simulink model "rolling_contact_test"  (R2026b)
settings: Solver=VariableStepAuto  StopTime=5
undefined symbols (not defined in the file): f_rr, k_contact, k_gx, k_gy, k_x, m_body, m_wheel, miu_p, miu_s, mu_slide, mu_stick, omega_rr_eps, r_wheel, sgn, v_c_max, v_gx_max, v_gy_max, vLimit, X, Y, Z
libraries: nesl_utility x19, sm_lib x18, simulink x7, simulink_extras x1
settings Model: Creator=h4nty  LastModifiedBy=h4nty
settings RTWCC: GPUComputeCapability=5.0
settings SimscapeCC: SimscapeUseEnergyAccounting=off

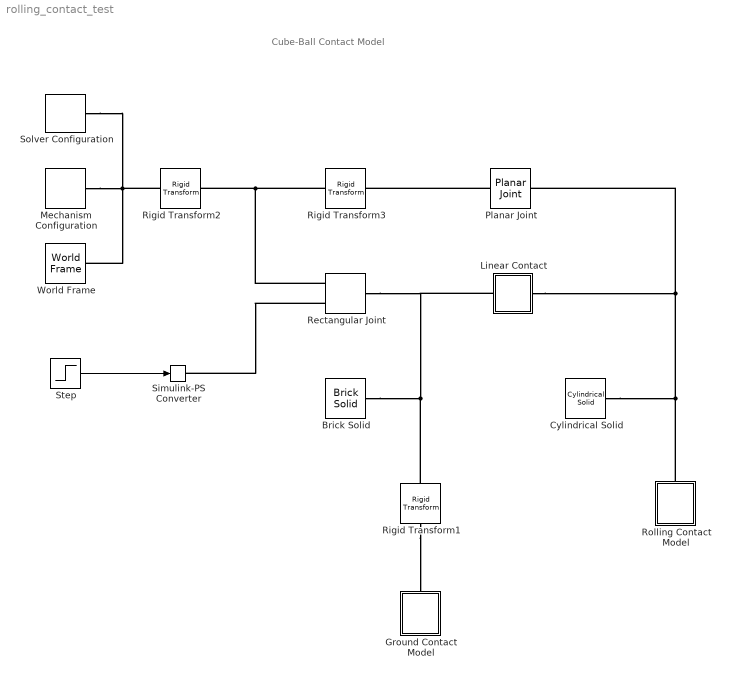
== system rolling_contact_test ==
  note: Cube-Ball Contact Model
  Brick Solid : sm_lib/Body Elements/Brick Solid  BrickDimensions=[1 1 1 ]  BrickDimensionsUnits=m  ExportEntireGeometry=off  InertiaType=CalculateFromGeometry  BasedOnType=Mass  Density=1000  DensityUnits=kg/m^3  Mass=m_body  MassUnits=kg  CenterOfMass=[0 0 0]  CenterOfMassUnits=m  MomentsOfInertia=[1 1 1]  MomentsOfInertiaUnits=kg*m^2  ProductsOfInertia=[0 0 0]  ProductsOfInertiaUnits=kg*m^2  GraphicType=FromGeometry  MarkerShape=Sphere  MarkerSize=10  GraphicVisPropType=SimpleVisualProperties  GraphicDiffuseColor=[0.5 0.5 0.5]  GraphicOpacity=1  GraphicSpecularColor=[0.5 0.5 0.5 1.0]  GraphicAmbientColor=[0.15 0.15 0.15 1.0]  GraphicEmissiveColor=[0.0 0.0 0.0 1.0]  GraphicShininess=75  DoExposeReferenceFrame=on  SerializedFrames=<Frames/>
  Cylindrical Solid : sm_lib/Body Elements/Cylindrical Solid  CylinderRadius=0.5  CylinderRadiusUnits=m  CylinderLength=1  CylinderLengthUnits=m  ExportEntireGeometry=off  InertiaType=CalculateFromGeometry  BasedOnType=Mass  Density=1000  DensityUnits=kg/m^3  Mass=m_wheel  MassUnits=kg  CenterOfMass=[0 0 0]  CenterOfMassUnits=m  MomentsOfInertia=[1 1 1]  MomentsOfInertiaUnits=kg*m^2  ProductsOfInertia=[0 0 0]  ProductsOfInertiaUnits=kg*m^2  GraphicType=FromGeometry  MarkerShape=Sphere  MarkerSize=10  GraphicVisPropType=SimpleVisualProperties  GraphicDiffuseColor=[0.5 0.5 0.5]  GraphicOpacity=1  GraphicSpecularColor=[0.5 0.5 0.5 1.0]  GraphicAmbientColor=[0.15 0.15 0.15 1.0]  GraphicEmissiveColor=[0.0 0.0 0.0 1.0]  GraphicShininess=75  DoExposeReferenceFrame=on  SerializedFrames=<Frames/>
  Ground Contact Model : Subsystem
  Linear Contact : Subsystem
  Mechanism Configuration : sm_lib/Utilities/Mechanism Configuration  UniformGravity=Constant  GravityVector=[0 -9.80665 0]  GravityVectorUnits=m/s^2  LinearizationDelta=0.001  JointModeTransitionNonlinearIterations=2
  Planar Joint : sm_lib/Joints/Planar Joint  JointMode=Normal  CompositeWrenchDir=FollowerOnBase  CompositeWrenchFrame=BaseFrame  SenseConstraintForce=off  SenseConstraintTorque=off  SenseTotalForce=off  SenseTotalTorque=off  PxPositionTargetSpecify=off  PxPositionTargetPriority=High  PxPositionTargetValue=0  PxPositionTargetValueUnits=m  PxVelocityTargetSpecify=off  PxVelocityTargetPriority=High  PxVelocityTargetValue=0  PxVelocityTargetValueUnits=m/s  PxEquilibriumPosition=0  PxEquilibriumPositionUnits=m  PxSpringStiffness=0  PxSpringStiffnessUnits=N/m  PxDampingCoefficient=0  PxDampingCoefficientUnits=N/(m/s)  PxLowerLimitSpecify=off  PxLowerLimitBound=-1  PxLowerLimitBoundUnits=m  PxLowerLimitStiffness=1e6  PxLowerLimitStiffnessUnits=N/m  PxLowerLimitDamping=1e3  PxLowerLimitDampingUnits=N/(m/s)  PxLowerLimitTransitionRegionWidth=1e-4  PxLowerLimitTransitionRegionWidthUnits=m  PxUpperLimitSpecify=off  PxUpperLimitBound=1  PxUpperLimitBoundUnits=m  PxUpperLimitStiffness=1e6  PxUpperLimitStiffnessUnits=N/m  PxUpperLimitDamping=1e3  PxUpperLimitDampingUnits=N/(m/s)  PxUpperLimitTransitionRegionWidth=1e-4  PxUpperLimitTransitionRegionWidthUnits=m  PxTorqueActuationMode=NoTorque  PxMotionActuationMode=ComputedMotion  PxSensePosition=off  PxSenseVelocity=off  PxSenseAcceleration=off  PxSenseTorqueForce=off  PxSenseLowerLimitTorqueForce=off  PxSenseUpperLimitTorqueForce=off  PyPositionTargetSpecify=off  PyPositionTargetPriority=High  PyPositionTargetValue=0  PyPositionTargetValueUnits=m  PyVelocityTargetSpecify=off  PyVelocityTargetPriority=High  PyVelocityTargetValue=0  PyVelocityTargetValueUnits=m/s  PyEquilibriumPosition=0  PyEquilibriumPositionUnits=m  PySpringStiffness=0  PySpringStiffnessUnits=N/m  PyDampingCoefficient=0  PyDampingCoefficientUnits=N/(m/s)  PyLowerLimitSpecify=off  PyLowerLimitBound=-1  PyLowerLimitBoundUnits=m  PyLowerLimitStiffness=1e6  PyLowerLimitStiffnessUnits=N/m  PyLowerLimitDamping=1e3  PyLowerLimitDampingUnits=N/(m/s)  PyLowerLimitTransitionRegionWidth=1e-4  PyLowerLimitTransitionRegionWidthUnits=m  PyUpperLimitSpecify=off  PyUpperLimitBound=1  PyUpperLimitBoundUnits=m  PyUpperLimitStiffness=1e6  PyUpperLimitStiffnessUnits=N/m  PyUpperLimitDamping=1e3  PyUpperLimitDampingUnits=N/(m/s)  PyUpperLimitTransitionRegionWidth=1e-4  PyUpperLimitTransitionRegionWidthUnits=m  PyTorqueActuationMode=NoTorque  PyMotionActuationMode=ComputedMotion  PySensePosition=off  PySenseVelocity=off  PySenseAcceleration=off  PySenseTorqueForce=off  PySenseLowerLimitTorqueForce=off  PySenseUpperLimitTorqueForce=off  RzPositionTargetSpecify=off  RzPositionTargetPriority=High  RzPositionTargetValue=0  RzPositionTargetValueUnits=deg  RzVelocityTargetSpecify=off  RzVelocityTargetPriority=High  RzVelocityTargetValue=0  RzVelocityTargetValueUnits=deg/s  RzEquilibriumPosition=0  RzEquilibriumPositionUnits=deg  RzSpringStiffness=0  RzSpringStiffnessUnits=N*m/deg  RzDampingCoefficient=0  RzDampingCoefficientUnits=N*m/(deg/s)  RzLowerLimitSpecify=off  RzLowerLimitBound=-90  RzLowerLimitBoundUnits=deg  RzLowerLimitStiffness=1e4  RzLowerLimitStiffnessUnits=N*m/deg  RzLowerLimitDamping=10  RzLowerLimitDampingUnits=N*m/(deg/s)  RzLowerLimitTransitionRegionWidth=0.1  RzLowerLimitTransitionRegionWidthUnits=deg  RzUpperLimitSpecify=off  RzUpperLimitBound=90  RzUpperLimitBoundUnits=deg  RzUpperLimitStiffness=1e4  RzUpperLimitStiffnessUnits=N*m/deg  RzUpperLimitDamping=10  RzUpperLimitDampingUnits=N*m/(deg/s)  RzUpperLimitTransitionRegionWidth=0.1  RzUpperLimitTransitionRegionWidthUnits=deg  RzTorqueActuationMode=NoTorque  RzMotionActuationMode=ComputedMotion  RzSensePosition=off  RzSenseVelocity=off  RzSenseAcceleration=off  RzSenseTorqueForce=off  RzSenseLowerLimitTorqueForce=off  RzSenseUpperLimitTorqueForce=off
  Rectangular Joint : sm_lib/Joints/Rectangular Joint  JointMode=Normal  CompositeWrenchDir=FollowerOnBase  CompositeWrenchFrame=BaseFrame  SenseConstraintForce=off  SenseConstraintTorque=off  SenseTotalForce=off  SenseTotalTorque=off  PxPositionTargetSpecify=off  PxPositionTargetPriority=High  PxPositionTargetValue=0  PxPositionTargetValueUnits=m  PxVelocityTargetSpecify=off  PxVelocityTargetPriority=High  PxVelocityTargetValue=0  PxVelocityTargetValueUnits=m/s  PxEquilibriumPosition=0  PxEquilibriumPositionUnits=m  PxSpringStiffness=0  PxSpringStiffnessUnits=N/m  PxDampingCoefficient=0  PxDampingCoefficientUnits=N/(m/s)  PxLowerLimitSpecify=off  PxLowerLimitBound=-1  PxLowerLimitBoundUnits=m  PxLowerLimitStiffness=1e6  PxLowerLimitStiffnessUnits=N/m  PxLowerLimitDamping=1e3  PxLowerLimitDampingUnits=N/(m/s)  PxLowerLimitTransitionRegionWidth=1e-4  PxLowerLimitTransitionRegionWidthUnits=m  PxUpperLimitSpecify=off  PxUpperLimitBound=1  PxUpperLimitBoundUnits=m  PxUpperLimitStiffness=1e6  PxUpperLimitStiffnessUnits=N/m  PxUpperLimitDamping=1e3  PxUpperLimitDampingUnits=N/(m/s)  PxUpperLimitTransitionRegionWidth=1e-4  PxUpperLimitTransitionRegionWidthUnits=m  PxTorqueActuationMode=InputTorque  PxMotionActuationMode=ComputedMotion  PxSensePosition=off  PxSenseVelocity=off  PxSenseAcceleration=off  PxSenseTorqueForce=off  PxSenseLowerLimitTorqueForce=off  PxSenseUpperLimitTorqueForce=off  PyPositionTargetSpecify=off  PyPositionTargetPriority=High  PyPositionTargetValue=0  PyPositionTargetValueUnits=m  PyVelocityTargetSpecify=off  PyVelocityTargetPriority=High  PyVelocityTargetValue=0  PyVelocityTargetValueUnits=m/s  PyEquilibriumPosition=0  PyEquilibriumPositionUnits=m  PySpringStiffness=0  PySpringStiffnessUnits=N/m  PyDampingCoefficient=0  PyDampingCoefficientUnits=N/(m/s)  PyLowerLimitSpecify=off  PyLowerLimitBound=-1  PyLowerLimitBoundUnits=m  PyLowerLimitStiffness=1e6  PyLowerLimitStiffnessUnits=N/m  PyLowerLimitDamping=1e3  PyLowerLimitDampingUnits=N/(m/s)  PyLowerLimitTransitionRegionWidth=1e-4  PyLowerLimitTransitionRegionWidthUnits=m  PyUpperLimitSpecify=off  PyUpperLimitBound=1  PyUpperLimitBoundUnits=m  PyUpperLimitStiffness=1e6  PyUpperLimitStiffnessUnits=N/m  PyUpperLimitDamping=1e3  PyUpperLimitDampingUnits=N/(m/s)  PyUpperLimitTransitionRegionWidth=1e-4  PyUpperLimitTransitionRegionWidthUnits=m  PyTorqueActuationMode=NoTorque  PyMotionActuationMode=ComputedMotion  PySensePosition=off  PySenseVelocity=off  PySenseAcceleration=off  PySenseTorqueForce=off  PySenseLowerLimitTorqueForce=off  PySenseUpperLimitTorqueForce=off
  Rigid Transform1 : sm_lib/Frames and Transforms/Rigid Transform  RotationMethod=None  FollAlignAxisA=+X  BaseAlignAxisA=+Y  FollAlignAxisB=+Y  BaseAlignAxisB=+Z  RotationStandardAxis=+Y  RotationAngle=-90  RotationAngleUnits=deg  RotationArbitraryAxis=[0 0 1]  RotationSequenceAxes=FollowerAxes  RotationSequence=XYX  RotationSequenceAngles=[0 0 0]  RotationSequenceAnglesUnits=deg  RotationMatrix=[1 0 0; 0 1 0; 0 0 1]  Quaternion=[1 0 0 0]  TranslationMethod=Cartesian  TranslationCartesianOffset=[0 -0.5 0]  TranslationCartesianOffsetUnits=m  TranslationStandardAxis=+X  TranslationStandardOffset=+0.5  TranslationStandardOffsetUnits=m  TranslationROffset=r_ball  TranslationROffsetUnits=m  TranslationThetaOffset=0  TranslationThetaOffsetUnits=deg  TranslationZOffset=0  TranslationZOffsetUnits=m
  Rigid Transform2 : sm_lib/Frames and Transforms/Rigid Transform  RotationMethod=None  FollAlignAxisA=+X  BaseAlignAxisA=+Y  FollAlignAxisB=+Y  BaseAlignAxisB=+Z  RotationStandardAxis=+Y  RotationAngle=90  RotationAngleUnits=deg  RotationArbitraryAxis=[0 0 1]  RotationSequenceAxes=FollowerAxes  RotationSequence=XYX  RotationSequenceAngles=[0 0 0]  RotationSequenceAnglesUnits=deg  RotationMatrix=[1 0 0; 0 1 0; 0 0 1]  Quaternion=[1 0 0 0]  TranslationMethod=Cartesian  TranslationCartesianOffset=[0 +0.5 0]  TranslationCartesianOffsetUnits=m  TranslationStandardAxis=+X  TranslationStandardOffset=+0.5  TranslationStandardOffsetUnits=m  TranslationROffset=r_ball  TranslationROffsetUnits=m  TranslationThetaOffset=0  TranslationThetaOffsetUnits=deg  TranslationZOffset=0  TranslationZOffsetUnits=m
  Rigid Transform3 : sm_lib/Frames and Transforms/Rigid Transform  RotationMethod=None  FollAlignAxisA=+X  BaseAlignAxisA=+Y  FollAlignAxisB=+Y  BaseAlignAxisB=+Z  RotationStandardAxis=+Y  RotationAngle=90  RotationAngleUnits=deg  RotationArbitraryAxis=[0 0 1]  RotationSequenceAxes=FollowerAxes  RotationSequence=XYX  RotationSequenceAngles=[0 0 0]  RotationSequenceAnglesUnits=deg  RotationMatrix=[1 0 0; 0 1 0; 0 0 1]  Quaternion=[1 0 0 0]  TranslationMethod=Cartesian  TranslationCartesianOffset=[2 0 0]  TranslationCartesianOffsetUnits=m  TranslationStandardAxis=+X  TranslationStandardOffset=+0.5  TranslationStandardOffsetUnits=m  TranslationROffset=r_ball  TranslationROffsetUnits=m  TranslationThetaOffset=0  TranslationThetaOffsetUnits=deg  TranslationZOffset=0  TranslationZOffsetUnits=m
  Rolling Contact Model : Subsystem
  Simulink-PS Converter : nesl_utility/Simulink-PS Converter  PhysicalDomain=network_engine_domain  SubClassName=ps_input  LeftPortType=input  RightPortType=output  PseudoPeriodic=off  Frequencies=[]  NoiseDistribution=none  NoiseParameters=[]  Unit=N  AffineConversion=off  FilteringAndDerivatives=provide  SimscapeFilterOrder=1  InputFilterTimeConstant=0.001  UdotUserProvided=0
  Solver Configuration : nesl_utility/Solver Configuration  PhysicalDomain=network_engine_domain  SubClassName=solver  LeftPortType=input  RightPortType=generic  Tones=[]  Harmonics=[]  SimulateNoise=off  Profile=off  UseLocalSampling=off  EnableSwitchedLinearOptims=on  FrequencyDomain=off  UseCCode=off  RelTol=0.001  AbsTol=0.001  MinStep=1e-09  ToWorkspace=off  RevertToSquareIcSolve=off  NumHomotopyIterations=100  PhasorMode=off  PhasorModeNumHarmonics=1  ConsistencySolver=NEWTON_FTOL  CanonicalOrdering=UNORDERED  OptimizeIntermediates=UNOPTIMIZED  MulticoreSolverChoice=BACKWARD_EULER  IndexReductionMethod=DerivativeReplacement  DoDC=off  ResidualTolerance=1e-09  ConsistencyTolSource=GLOBAL  ConsistencyAbsTol=0.001  ConsistencyRelTol=0.001  ConsistencyTolFactor=0.001  UseLocalSolver=off  LocalSolverChoice=NE_BACKWARD_EULER_ADVANCER  ResolveIndetEquations=on  FunctionEvalNumThread=1  LocalSolverSampleTime=0.001  DoFixedCost=off  MaxNonlinIter=3  MaxModeIter=2  ComputeImpulses=off  ImpulseIterations=2  LinearAlgebra=auto  LinearAlgebraNumThread=0  EquationFormulation=NE_TIME_EF  DelaysMemoryBudget=1024  AutomaticFiltering=on  FilteringTimeConstant=0.001  PartitionStorageMethod=AS_NEEDED  PartitionMemoryBudget=1024  PartitionMethod=BALANCED  MultibodyUseLocalSolver=off  MultibodyLocalSolverChoice=ODE1  MultibodyLocalSolverSampleTime=0.001
  Step : Step  InitialValue=100  FinalValue=0  SampleTime=0
  "World Frame " : sm_lib/Frames and Transforms/World Frame
  wires:
  Step/1 -> Simulink-PS Converter/1
  connections:
  Rigid Transform1/RConn1 -- Ground Contact Model/LConn1
  Solver Configuration/RConn1 -- "World Frame "/RConn1 -- Rigid Transform2/LConn1 -- Mechanism Configuration/RConn1
  Rectangular Joint/LConn1 -- Rigid Transform3/LConn1 -- Rigid Transform2/RConn1
  Rigid Transform1/LConn1 -- Linear Contact/LConn1 -- Rectangular Joint/RConn1 -- Brick Solid/RConn1
  Rectangular Joint/LConn2 -- Simulink-PS Converter/RConn1
  Planar Joint/LConn1 -- Rigid Transform3/RConn1
  Rolling Contact Model/LConn1 -- Cylindrical Solid/RConn1 -- Linear Contact/RConn1 -- Planar Joint/RConn1

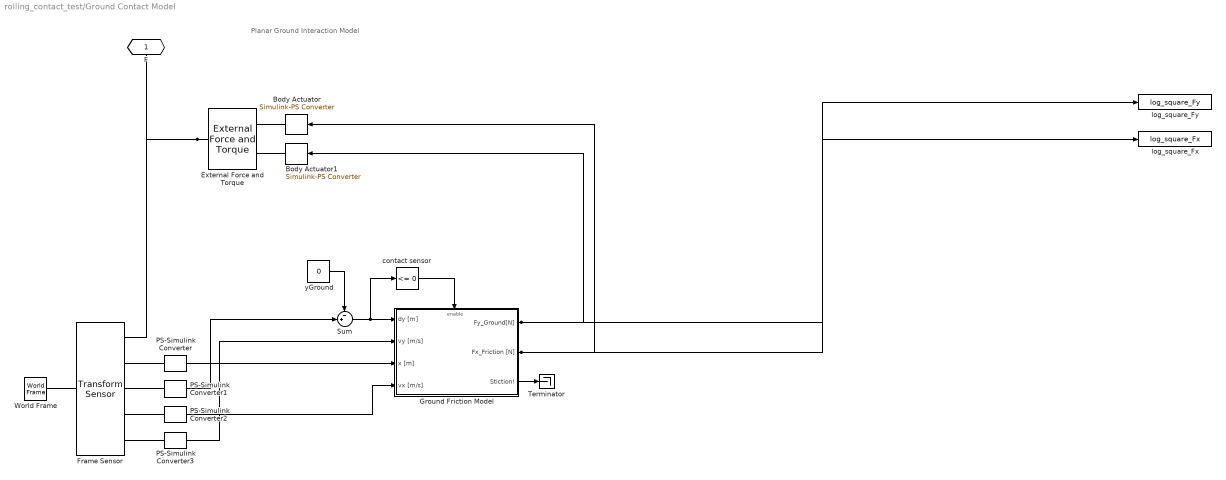
== system rolling_contact_test/Ground Contact Model ==
  note: Planar Ground Interaction Model
  " Body Actuator" : nesl_utility/Simulink-PS Converter  PhysicalDomain=network_engine_domain  SubClassName=ps_input  LeftPortType=input  RightPortType=output  PseudoPeriodic=off  Frequencies=[]  NoiseDistribution=none  NoiseParameters=[]  Unit=N  AffineConversion=off  FilteringAndDerivatives=zero  SimscapeFilterOrder=1  InputFilterTimeConstant=.001  UdotUserProvided=0
  " Body Actuator1" : nesl_utility/Simulink-PS Converter  PhysicalDomain=network_engine_domain  SubClassName=ps_input  LeftPortType=input  RightPortType=output  PseudoPeriodic=off  Frequencies=[]  NoiseDistribution=none  NoiseParameters=[]  Unit=N  AffineConversion=off  FilteringAndDerivatives=zero  SimscapeFilterOrder=1  InputFilterTimeConstant=.001  UdotUserProvided=0
  External Force and Torque : sm_lib/Forces and Torques/External Force and Torque  EnableForceX=on  EnableForceY=on  EnableForceZ=off  EnableForce=off  ForceResolutionFrame=World  EnableTorqueX=off  EnableTorqueY=off  EnableTorqueZ=off  EnableTorque=off  TorqueResolutionFrame=AttachedFrame
  Frame Sensor : sm_lib/Frames and Transforms/Transform Sensor  ObservationFrame=World  ExpressedInFrame=World  RotationSequence=XYX  SenseAngle=off  SenseAxis=off  SenseQ=off  SenseR=off  SenseRotationSequence=off  SenseOmegaX=off  SenseOmegaY=off  SenseOmegaZ=off  SenseOmega=off  SenseQDot=off  SenseRDot=off  SenseRotationSequenceDot=off  SenseAlphaX=off  SenseAlphaY=off  SenseAlphaZ=off  SenseAlpha=off  SenseQDDot=off  SenseRDDot=off  SenseX=on  SenseY=on  SenseZ=off  SenseXYZ=off  SenseRad=off  SenseAzim=off  SenseDist=off  SenseInc=off  SenseXDot=on  SenseYDot=on  SenseZDot=off  SenseXYZDot=off  SenseRadDot=off  SenseAzimDot=off  SenseDistDot=off  SenseIncDot=off  SenseXDDot=off  SenseYDDot=off  SenseZDDot=off  SenseXYZDDot=off  SenseRadDDot=off  SenseAzimDDot=off  SenseDistDDot=off  SenseIncDDot=off
  Ground Friction Model : Subsystem
  PS-Simulink Converter : nesl_utility/PS-Simulink Converter  PhysicalDomain=network_engine_domain  SubClassName=ps_output  LeftPortType=input  RightPortType=output  PseudoPeriodic=off  Frequencies=[]  VectorFormat=1-D array  Unit=m  AffineConversion=off
  PS-Simulink Converter1 : nesl_utility/PS-Simulink Converter  PhysicalDomain=network_engine_domain  SubClassName=ps_output  LeftPortType=input  RightPortType=output  PseudoPeriodic=off  Frequencies=[]  VectorFormat=1-D array  Unit=m  AffineConversion=off
  PS-Simulink Converter2 : nesl_utility/PS-Simulink Converter  PhysicalDomain=network_engine_domain  SubClassName=ps_output  LeftPortType=input  RightPortType=output  PseudoPeriodic=off  Frequencies=[]  VectorFormat=1-D array  Unit=m/s  AffineConversion=off
  PS-Simulink Converter3 : nesl_utility/PS-Simulink Converter  PhysicalDomain=network_engine_domain  SubClassName=ps_output  LeftPortType=input  RightPortType=output  PseudoPeriodic=off  Frequencies=[]  VectorFormat=1-D array  Unit=m/s  AffineConversion=off
  Sum : Sum  Inputs=-+|
  Terminator : Terminator
  World Frame : sm_lib/Frames and Transforms/World Frame
  contact sensor : simulink/Logic and Bit Operations/Compare To Zero  relop=<=  OutDataTypeStr=boolean
  log_square_Fx : ToWorkspace  VariableName=log_square_Fx  SaveFormat=Timeseries  SampleTime=-1
  log_square_Fy : ToWorkspace  VariableName=log_square_Fy  SaveFormat=Timeseries  SampleTime=-1
  yGround : Constant  Value=0
  F : PMIOPort  Side=Left
  wires:
  PS-Simulink Converter2/1 -> Ground Friction Model/4(vx [m/s])
  PS-Simulink Converter/1 -> Ground Friction Model/3(x [m])
  PS-Simulink Converter3/1 -> Ground Friction Model/2(vy [m/s])
  PS-Simulink Converter1/1 -> Sum/2
  Sum/1 -> contact sensor/1, Ground Friction Model/1(dy [m])
  yGround/1 -> Sum/1
  contact sensor/1 -> Ground Friction Model/Enable
  Ground Friction Model/1(Fy_Ground[N]) -> " Body Actuator1"/1, log_square_Fy/1
  Ground Friction Model/2(Fx_Friction [N]) -> " Body Actuator"/1, log_square_Fx/1
  Ground Friction Model/3(Stiction!) -> Terminator/1
  connections:
  World Frame/RConn1 -- Frame Sensor/LConn1
  PS-Simulink Converter2/LConn1 -- Frame Sensor/RConn4
  PS-Simulink Converter1/LConn1 -- Frame Sensor/RConn3
  Frame Sensor/RConn2 -- PS-Simulink Converter/LConn1
  PS-Simulink Converter3/LConn1 -- Frame Sensor/RConn5
  External Force and Torque/RConn1 -- Frame Sensor/RConn1 -- F/RConn1
  External Force and Torque/LConn2 -- " Body Actuator1"/RConn1
  External Force and Torque/LConn1 -- " Body Actuator"/RConn1

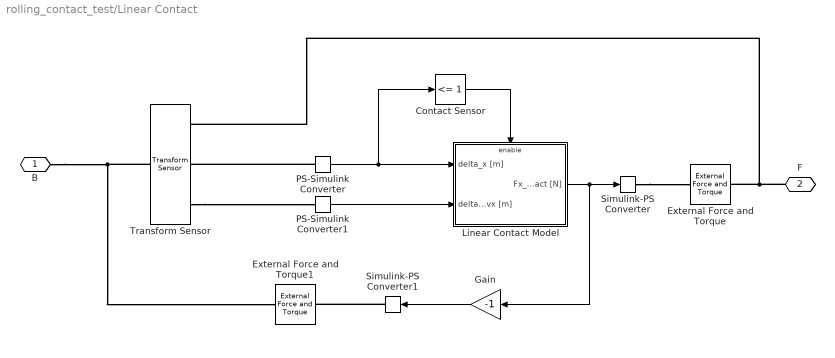
== system rolling_contact_test/Linear Contact ==
  Contact Sensor : simulink/Logic and Bit Operations/Compare To Constant  relop=<=  const=1  OutDataTypeStr=boolean  ZeroCross=off
  External Force and Torque : sm_lib/Forces and Torques/External Force and Torque  EnableForceX=on  EnableForceY=off  EnableForceZ=off  EnableForce=off  ForceResolutionFrame=AttachedFrame  EnableTorqueX=off  EnableTorqueY=off  EnableTorqueZ=off  EnableTorque=off  TorqueResolutionFrame=AttachedFrame
  External Force and Torque1 : sm_lib/Forces and Torques/External Force and Torque  EnableForceX=on  EnableForceY=off  EnableForceZ=off  EnableForce=off  ForceResolutionFrame=AttachedFrame  EnableTorqueX=off  EnableTorqueY=off  EnableTorqueZ=off  EnableTorque=off  TorqueResolutionFrame=AttachedFrame
  Gain : Gain  Gain=-1
  Linear Contact Model : Subsystem
  PS-Simulink Converter : nesl_utility/PS-Simulink Converter  PhysicalDomain=network_engine_domain  SubClassName=ps_output  LeftPortType=input  RightPortType=output  PseudoPeriodic=off  Frequencies=[]  VectorFormat=inherit  Unit=inherit  AffineConversion=off
  PS-Simulink Converter1 : nesl_utility/PS-Simulink Converter  PhysicalDomain=network_engine_domain  SubClassName=ps_output  LeftPortType=input  RightPortType=output  PseudoPeriodic=off  Frequencies=[]  VectorFormat=inherit  Unit=inherit  AffineConversion=off
  Simulink-PS Converter : nesl_utility/Simulink-PS Converter  PhysicalDomain=network_engine_domain  SubClassName=ps_input  LeftPortType=input  RightPortType=output  PseudoPeriodic=off  Frequencies=[]  NoiseDistribution=none  NoiseParameters=[]  Unit=1  AffineConversion=off  FilteringAndDerivatives=provide  SimscapeFilterOrder=1  InputFilterTimeConstant=0.001  UdotUserProvided=0
  Simulink-PS Converter1 : nesl_utility/Simulink-PS Converter  PhysicalDomain=network_engine_domain  SubClassName=ps_input  LeftPortType=input  RightPortType=output  PseudoPeriodic=off  Frequencies=[]  NoiseDistribution=none  NoiseParameters=[]  Unit=1  AffineConversion=off  FilteringAndDerivatives=provide  SimscapeFilterOrder=1  InputFilterTimeConstant=0.001  UdotUserProvided=0
  Transform Sensor : sm_lib/Frames and Transforms/Transform Sensor  ObservationFrame=World  ExpressedInFrame=World  RotationSequence=XYX  SenseAngle=off  SenseAxis=off  SenseQ=off  SenseR=off  SenseRotationSequence=off  SenseOmegaX=off  SenseOmegaY=off  SenseOmegaZ=off  SenseOmega=off  SenseQDot=off  SenseRDot=off  SenseRotationSequenceDot=off  SenseAlphaX=off  SenseAlphaY=off  SenseAlphaZ=off  SenseAlpha=off  SenseQDDot=off  SenseRDDot=off  SenseX=on  SenseY=off  SenseZ=off  SenseXYZ=off  SenseRad=off  SenseAzim=off  SenseDist=off  SenseInc=off  SenseXDot=on  SenseYDot=off  SenseZDot=off  SenseXYZDot=off  SenseRadDot=off  SenseAzimDot=off  SenseDistDot=off  SenseIncDot=off  SenseXDDot=off  SenseYDDot=off  SenseZDDot=off  SenseXYZDDot=off  SenseRadDDot=off  SenseAzimDDot=off  SenseDistDDot=off  SenseIncDDot=off
  B : PMIOPort  Side=Left
  F : PMIOPort  Port=2  Side=Right
  wires:
  PS-Simulink Converter/1 -> Linear Contact Model/1(delta_x [m]), Contact Sensor/1
  Contact Sensor/1 -> Linear Contact Model/Enable
  PS-Simulink Converter1/1 -> Linear Contact Model/2(delta_vx [m])
  Linear Contact Model/1(Fx_contact [N]) -> Gain/1, Simulink-PS Converter/1
  Gain/1 -> Simulink-PS Converter1/1
  connections:
  PS-Simulink Converter/LConn1 -- Transform Sensor/RConn2
  F/RConn1 -- Transform Sensor/RConn1 -- External Force and Torque/RConn1
  Transform Sensor/LConn1 -- B/RConn1 -- External Force and Torque1/RConn1
  Simulink-PS Converter/RConn1 -- External Force and Torque/LConn1
  Transform Sensor/RConn3 -- PS-Simulink Converter1/LConn1
  Simulink-PS Converter1/RConn1 -- External Force and Torque1/LConn1

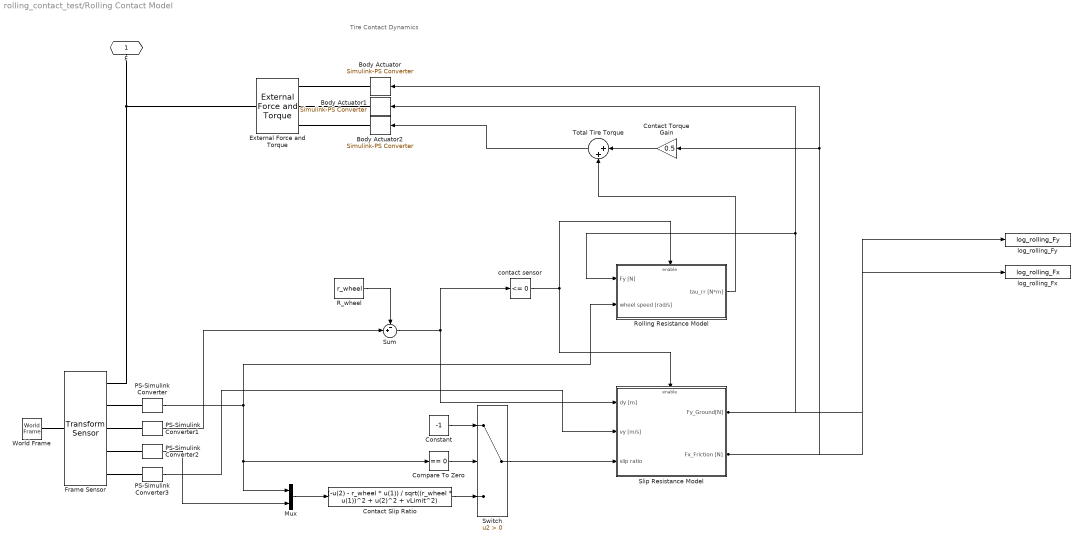
== system rolling_contact_test/Rolling Contact Model ==
  note: Tire Contact Dynamics
  " Body Actuator" : nesl_utility/Simulink-PS Converter  PhysicalDomain=network_engine_domain  SubClassName=ps_input  LeftPortType=input  RightPortType=output  PseudoPeriodic=off  Frequencies=[]  NoiseDistribution=none  NoiseParameters=[]  Unit=N  AffineConversion=off  FilteringAndDerivatives=zero  SimscapeFilterOrder=1  InputFilterTimeConstant=.001  UdotUserProvided=0
  " Body Actuator1" : nesl_utility/Simulink-PS Converter  PhysicalDomain=network_engine_domain  SubClassName=ps_input  LeftPortType=input  RightPortType=output  PseudoPeriodic=off  Frequencies=[]  NoiseDistribution=none  NoiseParameters=[]  Unit=N  AffineConversion=off  FilteringAndDerivatives=zero  SimscapeFilterOrder=1  InputFilterTimeConstant=.001  UdotUserProvided=0
  " Body Actuator2" : nesl_utility/Simulink-PS Converter  PhysicalDomain=network_engine_domain  SubClassName=ps_input  LeftPortType=input  RightPortType=output  PseudoPeriodic=off  Frequencies=[]  NoiseDistribution=none  NoiseParameters=[]  Unit=N*m  AffineConversion=off  FilteringAndDerivatives=zero  SimscapeFilterOrder=1  InputFilterTimeConstant=.001  UdotUserProvided=0
  Compare To Zero : simulink/Logic and Bit Operations/Compare To Zero  relop===  OutDataTypeStr=boolean
  Constant : Constant  Value=-1
  Contact Slip Ratio : Fcn  Expr=(-u(2) - r_wheel * u(1)) / sqrt((r_wheel * u(1))^2 + u(2)^2 + vLimit^2)
  Contact Torque Gain : Gain  Gain=0.5
  External Force and Torque : sm_lib/Forces and Torques/External Force and Torque  EnableForceX=on  EnableForceY=on  EnableForceZ=off  EnableForce=off  ForceResolutionFrame=World  EnableTorqueX=off  EnableTorqueY=off  EnableTorqueZ=on  EnableTorque=off  TorqueResolutionFrame=AttachedFrame
  Frame Sensor : sm_lib/Frames and Transforms/Transform Sensor  ObservationFrame=World  ExpressedInFrame=World  RotationSequence=XYX  SenseAngle=off  SenseAxis=off  SenseQ=off  SenseR=off  SenseRotationSequence=off  SenseOmegaX=off  SenseOmegaY=off  SenseOmegaZ=on  SenseOmega=off  SenseQDot=off  SenseRDot=off  SenseRotationSequenceDot=off  SenseAlphaX=off  SenseAlphaY=off  SenseAlphaZ=off  SenseAlpha=off  SenseQDDot=off  SenseRDDot=off  SenseX=off  SenseY=on  SenseZ=off  SenseXYZ=off  SenseRad=off  SenseAzim=off  SenseDist=off  SenseInc=off  SenseXDot=on  SenseYDot=on  SenseZDot=off  SenseXYZDot=off  SenseRadDot=off  SenseAzimDot=off  SenseDistDot=off  SenseIncDot=off  SenseXDDot=off  SenseYDDot=off  SenseZDDot=off  SenseXYZDDot=off  SenseRadDDot=off  SenseAzimDDot=off  SenseDistDDot=off  SenseIncDDot=off
  Mux : Mux  Inputs=2
  PS-Simulink Converter : nesl_utility/PS-Simulink Converter  PhysicalDomain=network_engine_domain  SubClassName=ps_output  LeftPortType=input  RightPortType=output  PseudoPeriodic=off  Frequencies=[]  VectorFormat=1-D array  Unit=rad/s  AffineConversion=off
  PS-Simulink Converter1 : nesl_utility/PS-Simulink Converter  PhysicalDomain=network_engine_domain  SubClassName=ps_output  LeftPortType=input  RightPortType=output  PseudoPeriodic=off  Frequencies=[]  VectorFormat=1-D array  Unit=m  AffineConversion=off
  PS-Simulink Converter2 : nesl_utility/PS-Simulink Converter  PhysicalDomain=network_engine_domain  SubClassName=ps_output  LeftPortType=input  RightPortType=output  PseudoPeriodic=off  Frequencies=[]  VectorFormat=1-D array  Unit=m/s  AffineConversion=off
  PS-Simulink Converter3 : nesl_utility/PS-Simulink Converter  PhysicalDomain=network_engine_domain  SubClassName=ps_output  LeftPortType=input  RightPortType=output  PseudoPeriodic=off  Frequencies=[]  VectorFormat=1-D array  Unit=m/s  AffineConversion=off
  R_wheel : Constant  Value=r_wheel
  Rolling Resistance Model : Subsystem
  Slip Resistance Model : Subsystem
  Sum : Sum  Inputs=-+|
  Switch : Switch  Criteria=u2 > Threshold  SaturateOnIntegerOverflow=off  InputSameDT=off
  Total Tire Torque : Sum  Inputs=|++
  World Frame : sm_lib/Frames and Transforms/World Frame
  contact sensor : simulink/Logic and Bit Operations/Compare To Zero  relop=<=  OutDataTypeStr=boolean
  log_rolling_Fx : ToWorkspace  VariableName=log_rolling_Fx  SaveFormat=Timeseries  SampleTime=-1
  log_rolling_Fy : ToWorkspace  VariableName=log_rolling_Fy  SaveFormat=Timeseries  SampleTime=-1
  F : PMIOPort  Side=Left
  wires:
  R_wheel/1 -> Sum/1
  Sum/1 -> contact sensor/1, Slip Resistance Model/1(dy [m])
  PS-Simulink Converter/1 -> Rolling Resistance Model/2(wheel speed [rad/s]), Mux/1, Compare To Zero/1
  Mux/1 -> Contact Slip Ratio/1
  PS-Simulink Converter1/1 -> Sum/2
  PS-Simulink Converter2/1 -> Mux/2
  Slip Resistance Model/1(Fy_Ground[N]) -> Rolling Resistance Model/1(Fy [N]), " Body Actuator1"/1, log_rolling_Fy/1
  Slip Resistance Model/2(Fx_Friction [N]) -> Contact Torque Gain/1, " Body Actuator"/1, log_rolling_Fx/1
  contact sensor/1 -> Slip Resistance Model/Enable, Rolling Resistance Model/Enable
  PS-Simulink Converter3/1 -> Slip Resistance Model/2(vy [m/s])
  Switch/1 -> Slip Resistance Model/3(slip ratio)
  Contact Slip Ratio/1 -> Switch/3
  Compare To Zero/1 -> Switch/2
  Constant/1 -> Switch/1
  Contact Torque Gain/1 -> Total Tire Torque/1
  Total Tire Torque/1 -> " Body Actuator2"/1
  Rolling Resistance Model/1(tau_rr [N*m]) -> Total Tire Torque/2
  connections:
  External Force and Torque/LConn1 -- " Body Actuator"/RConn1
  " Body Actuator1"/RConn1 -- External Force and Torque/LConn2
  F/RConn1 -- Frame Sensor/RConn1 -- External Force and Torque/RConn1
  PS-Simulink Converter3/LConn1 -- Frame Sensor/RConn5
  Frame Sensor/RConn2 -- PS-Simulink Converter/LConn1
  PS-Simulink Converter1/LConn1 -- Frame Sensor/RConn3
  PS-Simulink Converter2/LConn1 -- Frame Sensor/RConn4
  World Frame/RConn1 -- Frame Sensor/LConn1
  " Body Actuator2"/RConn1 -- External Force and Torque/LConn3

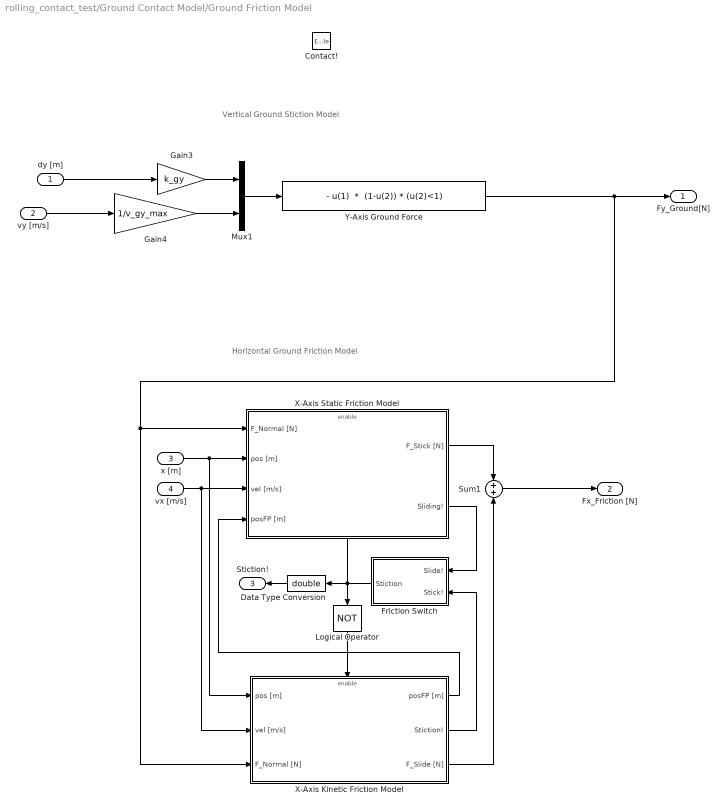
== system rolling_contact_test/Ground Contact Model/Ground Friction Model ==
  note: Horizontal Ground Friction Model
  note: Vertical Ground Stiction Model
  dy [m] : Inport
  vy [m/s] : Inport  Port=2
  x [m] : Inport  Port=3
  vx [m/s] : Inport  Port=4
  Contact! : EnablePort  StatesWhenEnabling=reset
  Data Type Conversion : DataTypeConversion  OutDataTypeStr=double  SaturateOnIntegerOverflow=off  RndMeth=Floor
  Friction Switch : Subsystem
  Gain3 : Gain  Gain=k_gy
  Gain4 : Gain  Gain=1/v_gy_max
  Logical Operator : Logic  Operator=NOT  AllPortsSameDT=off  OutDataTypeStr=boolean
  Mux1 : Mux  Inputs=2
  Sum1 : Sum
  X-Axis Kinetic Friction Model : Subsystem
  X-Axis Static Friction Model : Subsystem
  Y-Axis Ground Force : Fcn  Expr="- u(1)  *  (1-u(2)) * (u(2)<1)"
  Fy_Ground[N] : Outport  OutputWhenDisabled=reset  InitialOutput=0
      settings: AttributesFormatString=initial = '%<InitialOutput>'\nwhen disabled = '%<OutputWhenDisabled>'
  Fx_Friction [N] : Outport  Port=2  OutputWhenDisabled=reset  InitialOutput=0
      settings: AttributesFormatString=initial = '%<InitialOutput>'\nwhen\ndisabled\n'%<OutputWhenDisabled>'
  Stiction! : Outport  Port=3  OutputWhenDisabled=reset  InitialOutput=0
      settings: AttributesFormatString=initial = '%<InitialOutput>'\nwhen\ndisabled\n'%<OutputWhenDisabled>'
  wires:
  Y-Axis Ground Force/1 -> X-Axis Static Friction Model/1(F_Normal [N]), X-Axis Kinetic Friction Model/3(F_Normal [N]), Fy_Ground[N]/1
  dy [m]/1 -> Gain3/1
  vy [m/s]/1 -> Gain4/1
  x [m]/1 -> X-Axis Static Friction Model/2(pos [m]), X-Axis Kinetic Friction Model/1(pos [m])
  vx [m/s]/1 -> X-Axis Static Friction Model/3(vel [m/s]), X-Axis Kinetic Friction Model/2(vel [m/s])
  X-Axis Kinetic Friction Model/1(posFP [m]) -> X-Axis Static Friction Model/4(posFP [m])
  X-Axis Kinetic Friction Model/3(F_Slide [N]) -> Sum1/2
  X-Axis Static Friction Model/1(F_Stick [N]) -> Sum1/1
  Sum1/1 -> Fx_Friction [N]/1
  Friction Switch/1(Stiction) -> X-Axis Static Friction Model/Enable, Logical Operator/1, Data Type Conversion/1
  X-Axis Static Friction Model/2(Sliding!) -> Friction Switch/1(Slide!)
  X-Axis Kinetic Friction Model/2(Stiction!) -> Friction Switch/2(Stick!)
  Logical Operator/1 -> X-Axis Kinetic Friction Model/Enable
  Data Type Conversion/1 -> Stiction!/1
  Mux1/1 -> Y-Axis Ground Force/1
  Gain3/1 -> Mux1/1
  Gain4/1 -> Mux1/2

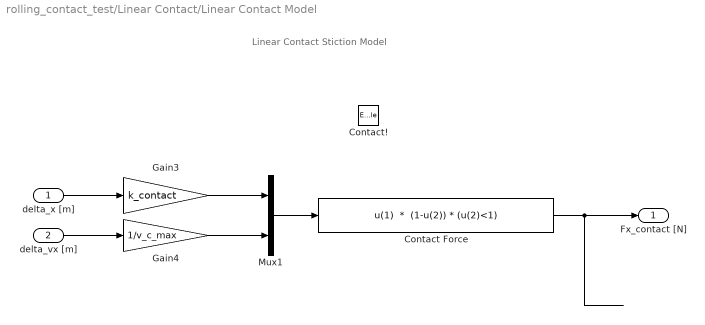
== system rolling_contact_test/Linear Contact/Linear Contact Model ==
  note: Linear Contact Stiction Model
  delta_x [m] : Inport
  delta_vx [m] : Inport  Port=2
  Contact! : EnablePort  StatesWhenEnabling=reset
  Contact Force : Fcn  Expr="u(1)  *  (1-u(2)) * (u(2)<1)"
  Gain3 : Gain  Gain=k_contact
  Gain4 : Gain  Gain=1/v_c_max
  Mux1 : Mux  Inputs=2
  Fx_contact [N] : Outport  OutputWhenDisabled=reset  InitialOutput=0
  wires:
  Contact Force/1 -> Fx_contact [N]/1
  delta_vx [m]/1 -> Gain4/1
  delta_x [m]/1 -> Gain3/1
  Mux1/1 -> Contact Force/1
  Gain4/1 -> Mux1/2
  Gain3/1 -> Mux1/1

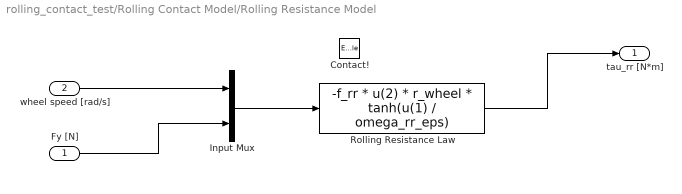
== system rolling_contact_test/Rolling Contact Model/Rolling Resistance Model ==
  Fy [N] : Inport
  wheel speed [rad/s] : Inport  Port=2
  Contact! : EnablePort
  Input Mux : Mux  Inputs=2
  Rolling Resistance Law : Fcn  Expr=-f_rr * u(2) * r_wheel * tanh(u(1) / omega_rr_eps)
  tau_rr [N*m] : Outport
  wires:
  wheel speed [rad/s]/1 -> Input Mux/1
  Fy [N]/1 -> Input Mux/2
  Rolling Resistance Law/1 -> tau_rr [N*m]/1
  Input Mux/1 -> Rolling Resistance Law/1

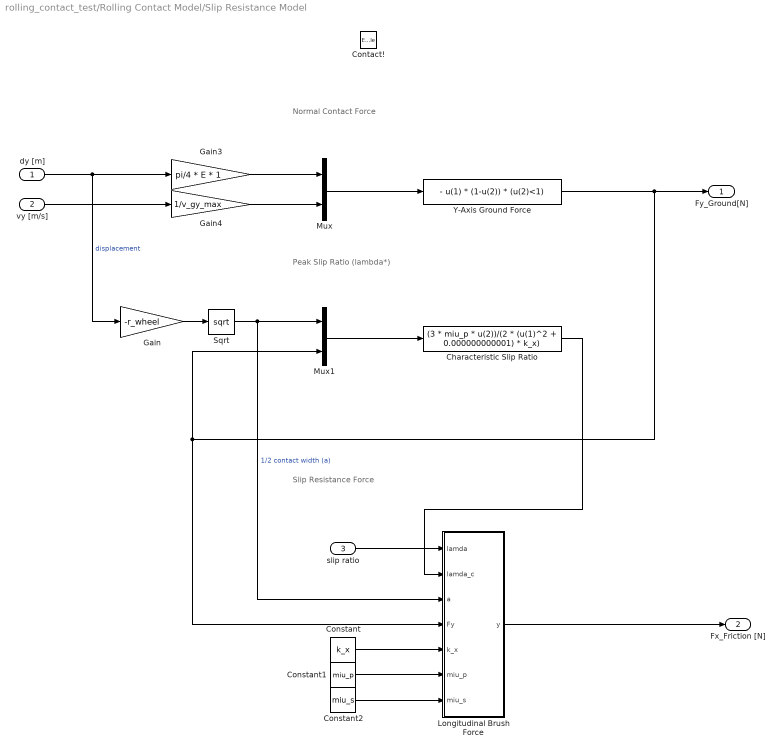
== system rolling_contact_test/Rolling Contact Model/Slip Resistance Model ==
  note: Normal Contact Force
  note: Slip Resistance Force
  note: Peak Slip Ratio (lambda*)
  dy [m] : Inport
  vy [m/s] : Inport  Port=2
  slip ratio : Inport  Port=3
  Contact! : EnablePort  StatesWhenEnabling=reset
  Characteristic Slip Ratio : Fcn  Expr=(3 * miu_p * u(2))/(2 * (u(1)^2 + 0.000000000001) * k_x)
  Constant : Constant  Value=k_x
  Constant1 : Constant  Value=miu_p
  Constant2 : Constant  Value=miu_s
  Gain : Gain  Gain=-r_wheel
  Gain3 : Gain  Gain=pi/4 * E * 1
  Gain4 : Gain  Gain=1/v_gy_max
  Longitudinal Brush Force : MATLAB Function  TreatAsAtomicUnit=on
  Mux : Mux  Inputs=2
  Mux1 : Mux  Inputs=2
  Sqrt : Sqrt
  Y-Axis Ground Force : Fcn  Expr=- u(1) * (1-u(2)) * (u(2)<1)
  Fy_Ground[N] : Outport  OutputWhenDisabled=reset  InitialOutput=0
      settings: AttributesFormatString=initial = '%<InitialOutput>'\nwhen disabled = '%<OutputWhenDisabled>'
  Fx_Friction [N] : Outport  Port=2  OutputWhenDisabled=reset  InitialOutput=0
      settings: AttributesFormatString=initial = '%<InitialOutput>'\nwhen\ndisabled\n'%<OutputWhenDisabled>'
  wires:
  Gain4/1 -> Mux/2
  dy [m]/1 -> Gain3/1, Gain/1  "displacement"
  Mux/1 -> Y-Axis Ground Force/1
  vy [m/s]/1 -> Gain4/1
  Gain3/1 -> Mux/1
  Gain/1 -> Sqrt/1
  Sqrt/1 -> Longitudinal Brush Force/3(a), Mux1/1  "1/2 contact width (a)"
  Mux1/1 -> Characteristic Slip Ratio/1
  Y-Axis Ground Force/1 -> Fy_Ground[N]/1, Longitudinal Brush Force/4(Fy), Mux1/2
  slip ratio/1 -> Longitudinal Brush Force/1(lamda)
  Characteristic Slip Ratio/1 -> Longitudinal Brush Force/2(lamda_c)
  Constant/1 -> Longitudinal Brush Force/5(k_x)
  Constant1/1 -> Longitudinal Brush Force/6(miu_p)
  Constant2/1 -> Longitudinal Brush Force/7(miu_s)
  Longitudinal Brush Force/1(y) -> Fx_Friction [N]/1

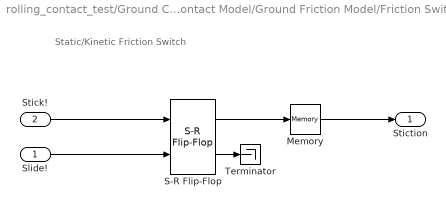
== system rolling_contact_test/Ground Contact Model/Ground Friction Model/Friction Switch ==
  note: Static/Kinetic Friction Switch
  Slide! : Inport
  Stick! : Inport  Port=2
  Memory : Memory
  S-R Flip-Flop : simulink_extras/Flip Flops/S-R Flip-Flop  initial_condition=1
  Terminator : Terminator
  Stiction : Outport
  wires:
  S-R Flip-Flop/1 -> Memory/1
  S-R Flip-Flop/2 -> Terminator/1
  Stick!/1 -> S-R Flip-Flop/1
  Slide!/1 -> S-R Flip-Flop/2
  Memory/1 -> Stiction/1

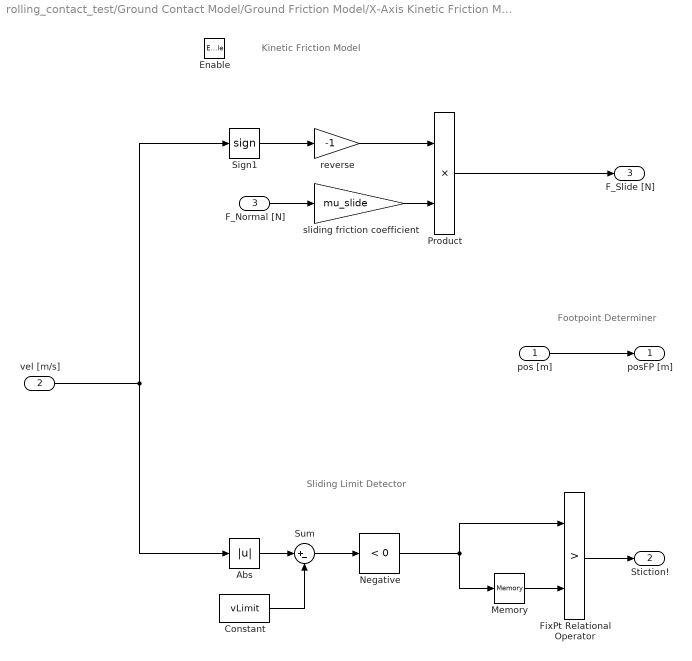
== system rolling_contact_test/Ground Contact Model/Ground Friction Model/X-Axis Kinetic Friction Model ==
  note: Kinetic Friction Model
  note: Footpoint Determiner
  note: Sliding Limit Detector
  pos [m] : Inport
  vel [m/s] : Inport  Port=2
  F_Normal [N] : Inport  Port=3
  Enable : EnablePort  StatesWhenEnabling=reset  ZeroCross=off
  Abs : Abs  SaturateOnIntegerOverflow=off
  Constant : Constant  Value=vLimit
  FixPt Relational Operator : RelationalOperator  Operator=>  OutDataTypeStr=boolean  ZeroCross=off  InputSameDT=off
  Memory : Memory
  Negative : simulink/Logic and Bit Operations/Compare To Zero  relop=<  OutDataTypeStr=boolean
  Product : Product  RndMeth=Zero
  Sign1 : Signum
  Sum : Sum  Inputs=|+-
  reverse : Gain  Gain=-1
  sliding friction coefficient : Gain  Gain=mu_slide
  posFP [m] : Outport  InitialOutput=0
      settings: AttributesFormatString=initial = '%<InitialOutput>'\nwhen disabled = '%<OutputWhenDisabled>'
  Stiction! : Outport  Port=2  OutputWhenDisabled=reset  InitialOutput=0
      settings: AttributesFormatString=initial = '%<InitialOutput>'\nwhen disabled = '%<OutputWhenDisabled>'
  F_Slide [N] : Outport  Port=3  OutputWhenDisabled=reset  InitialOutput=0
      settings: AttributesFormatString=initial = '%<InitialOutput>'\nwhen disabled = '%<OutputWhenDisabled>'
  wires:
  reverse/1 -> Product/1
  F_Normal [N]/1 -> sliding friction coefficient/1
  vel [m/s]/1 -> Sign1/1, Abs/1
  pos [m]/1 -> posFP [m]/1
  Product/1 -> F_Slide [N]/1
  sliding friction coefficient/1 -> Product/2
  Sign1/1 -> reverse/1
  FixPt Relational Operator/1 -> Stiction!/1
  Memory/1 -> FixPt Relational Operator/2
  Negative/1 -> FixPt Relational Operator/1, Memory/1
  Abs/1 -> Sum/1
  Sum/1 -> Negative/1
  Constant/1 -> Sum/2

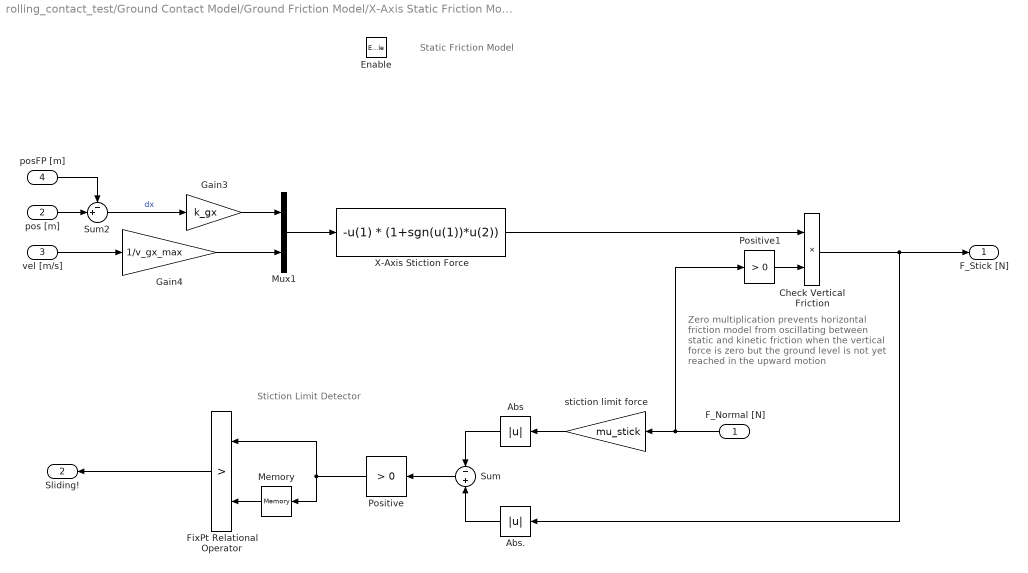
== system rolling_contact_test/Ground Contact Model/Ground Friction Model/X-Axis Static Friction Model ==
  note: Zero multiplication prevents
      | horizontal friction model from
      | oscillating between static and kinetic
      | friction when the vertical force is zero but
      | the ground level is not yet reached
      | in the upward motion
  note: Stiction Limit Detector
  note: Static Friction Model
  F_Normal [N] : Inport
  pos [m] : Inport  Port=2
  vel [m/s] : Inport  Port=3
  posFP [m] : Inport  Port=4
  Enable : EnablePort  StatesWhenEnabling=reset  ZeroCross=off
  Abs : Abs  SaturateOnIntegerOverflow=off
  Abs. : Abs  SaturateOnIntegerOverflow=off
  Check Vertical Friction : Product  RndMeth=Zero
  FixPt Relational Operator : RelationalOperator  Operator=>  OutDataTypeStr=boolean  ZeroCross=off  InputSameDT=off
  Gain3 : Gain  Gain=k_gx
  Gain4 : Gain  Gain=1/v_gx_max
  Memory : Memory
  Mux1 : Mux  Inputs=2
  Positive : simulink/Logic and Bit Operations/Compare To Zero  relop=>  OutDataTypeStr=boolean
  Positive1 : simulink/Logic and Bit Operations/Compare To Zero  relop=>  OutDataTypeStr=boolean
  Sum : Sum  Inputs=-+
  Sum2 : Sum  Inputs=-+|
  X-Axis Stiction Force : Fcn  Expr=-u(1) * (1+sgn(u(1))*u(2))
  stiction limit force : Gain  Gain=mu_stick
  F_Stick [N] : Outport  OutputWhenDisabled=reset  InitialOutput=0
      settings: AttributesFormatString=when disabled: %<OutputWhenDisabled>\ninitial: %<InitialOutput>
  Sliding! : Outport  Port=2  OutputWhenDisabled=reset  InitialOutput=0
      settings: AttributesFormatString=when disabled: %<OutputWhenDisabled>\ninitial: %<InitialOutput>
  wires:
  Check Vertical Friction/1 -> Abs./1, F_Stick [N]/1
  Positive1/1 -> Check Vertical Friction/2
  X-Axis Stiction Force/1 -> Check Vertical Friction/1
  stiction limit force/1 -> Abs/1
  Abs/1 -> Sum/1
  FixPt Relational Operator/1 -> Sliding!/1
  Gain4/1 -> Mux1/2
  Gain3/1 -> Mux1/1
  Mux1/1 -> X-Axis Stiction Force/1
  Abs./1 -> Sum/2
  Positive/1 -> Memory/1, FixPt Relational Operator/1
  Memory/1 -> FixPt Relational Operator/2
  Sum/1 -> Positive/1
  vel [m/s]/1 -> Gain4/1
  posFP [m]/1 -> Sum2/1
  pos [m]/1 -> Sum2/2
  Sum2/1 -> Gain3/1  "dx"
  F_Normal [N]/1 -> Positive1/1, stiction limit force/1

== matlab function rolling_contact_test/Rolling Contact Model/Slip Resistance Model/Longitudinal Brush Force ==
  data: lamda input; y output; lamda_c input; a input; Fy input; k_x input; miu_p input; miu_s input
function y = fcn(lamda, lamda_c, a, Fy, k_x, miu_p, miu_s)

slip_direction = sign(lamda);
slip_magnitude = abs(lamda);

if slip_magnitude <= lamda_c
    force_magnitude = 2 * a^2 * k_x * slip_magnitude * (1 - slip_magnitude / lamda_c) + miu_p * Fy * (slip_magnitude / lamda_c)^2 * (3 - 2 * slip_magnitude / lamda_c);
elseif slip_magnitude < 1
    force_magnitude = Fy * (miu_p + (miu_s - miu_p) * (slip_magnitude - lamda_c) / (1 - lamda_c));
else
    force_magnitude = miu_s * Fy;
end

y = slip_direction * force_magnitude;
